simulink model "Combined_MiniHex_Simulation"  (R2023b)
settings: Solver=VariableStepAuto  StartTime=0.0  StopTime=38  RelTol=1e-3
InitFcn:
  | addpath(genpath(pwd));
  | disp('✅ InitFcn executed');
  | Combined_Assembly_DataFile;  % Run the data file script to load smiData
model workspace: external: MAT-File C:\Users\amine\OneDrive - TUM\Desktop\Bachelor Thesis\SIMSCAPE\Simscape files\slprj\sim\varcache\Assembly_For_Simscape\varInfo.mat (data not in the file)
undefined symbols (not defined in the file or in its folder): sigbuilder_block, smiData, smiData_Upperstage, X, Y, Z
libraries: sm_lib x122, nesl_utility x35
(part 5 of 5)

== system Combined_MiniHex_Simulation/Project_MiniHex/Lower Stage (Stewart_Platform)/Horn-BallJoint-Rod-BallJoint 6/Rod_1_RIGID ==
  ReferenceFrame : sm_lib/Frames and Transforms/Reference Frame
  Solid : sm_lib/Body Elements/File Solid  ExtGeomFileName=Rod_Default_sldprt.STEP  UnitType=FromFile  ExtGeomFileUnits=m  StepReaderType=HEX  ExportConvexHullGeometry=off  InertiaType=Custom  Mass=smiData_Upperstage.Solid(3).mass  MassUnits=kg  CenterOfMass=smiData_Upperstage.Solid(3).CoM  CenterOfMassUnits=m  MomentsOfInertia=smiData_Upperstage.Solid(3).MoI  MomentsOfInertiaUnits=kg*m^2  ProductsOfInertia=smiData_Upperstage.Solid(3).PoI  ProductsOfInertiaUnits=kg*m^2  BasedOnType=DensityFromFile  Density=1000  DensityUnits=kg/m^3  DoExposeReferenceFrame=on  SerializedFrames=<Frames><Frame><Id>Frame1</Id><Value><Name>F1</Name><Origin><Source>GeometricFeature</Source><FeatureName>planar surface 4</FeatureName></Origin><PrimaryAxis><DefinedDirection>-Z</DefinedDirection><Source>GeometricFeature</Source><SourceDirection>+Z</SourceDirection><FeatureName>planar surface 4</FeatureName></PrimaryAxis><SecondaryAxis><DefinedDirection>+X</DefinedDirection><Source>ReferenceFrame</Source><SourceDirection>+X</SourceDirection><FeatureName></FeatureName></SecondaryAxis></Value></Frame><Frame><Id>Frame2</Id><Value><Name>F2</Name><Origin><Source>GeometricFeature</Source><FeatureName>planar surface 3</FeatureName></Origin><PrimaryAxis><DefinedDirection>-Z</DefinedDirection><Source>CenterOfMassFrame</Source><SourceDirection>+Y</SourceDirection><FeatureName></FeatureName></PrimaryAxis><SecondaryAxis><DefinedDirection>+Y</DefinedDirection><Source>CenterOfMassFrame</Source><SourceDirection>+Z</SourceDirection><FeatureName></FeatureName></SecondaryAxis></Value></Frame></Frames>  GraphicType=FromGeometry  MarkerShape=Sphere  MarkerSize=10  GraphicVisPropType=SimpleVisualProperties  GraphicDiffuseColor=smiData.Solid(3).color  GraphicSpecularColor=[0.5 0.5 0.5 1.0]  GraphicAmbientColor=[0.15 0.15 0.15 1.0]  GraphicEmissiveColor=[0.0 0.0 0.0 1.0]  GraphicShininess=75  GraphicOpacity=smiData.Solid(3).opacity
  F : PMIOPort  Side=Left
  F1 : PMIOPort  Port=2  Side=Right
  connections:
  ReferenceFrame/RConn1 -- Solid/RConn1
  Solid/LConn1 -- F/RConn1
  Solid/LConn2 -- F1/RConn1

== matlab function Combined_MiniHex_Simulation/Project_MiniHex/Servo_Angles ==
  data: roll input; servoAngles output; pitch input; yaw input; x input; y input; z input
function servoAngles = stewartBlock(roll, pitch, yaw, x, y, z)
%#codegen

pose = [roll, pitch, yaw, x, y, z];
servoAngles = stewartIK(pose);
servoAngles = reshape(servoAngles, [6, 1]);
end

== matlab function Combined_MiniHex_Simulation/Project_MiniHex/Uppe_Stage_Servo_Inputs/MATLAB Function1 ==
  data: t input; y output
function y = fcn(t)
  A = deg2rad(30);  % 30° in radians
  f = 0.1;            % Frequency in Hz
  y = A * sin(2*pi*f*t)+pi/2;
end

== matlab function Combined_MiniHex_Simulation/Project_MiniHex/Uppe_Stage_Servo_Inputs/MATLAB Function4 ==
  data: t input; y output
function y = fcn(t)
  A = deg2rad(30);  % 30° in radians
  f = 0.1;            % Frequency in Hz
  y = A * sin(2*pi*f*t)+pi/2;
end

== matlab function Combined_MiniHex_Simulation/Project_MiniHex/Uppe_Stage_Servo_Inputs/MATLAB Function3 ==
  data: t input; y output
function y = fcn(t)
  A = deg2rad(30);  % 30° in radians
  f = 0.1;            % Frequency in Hz
  y = A * sin(2*pi*f*t);
end
